simulink model "StampFly_StudentBlocks"  (R2026b)
settings: Solver=VariableStepAuto
undefined symbols (not defined in the file): Bottom, Official
(part 1 of 6)
settings Model: Creator=tyasukaw  LastModifiedBy=tyasukaw

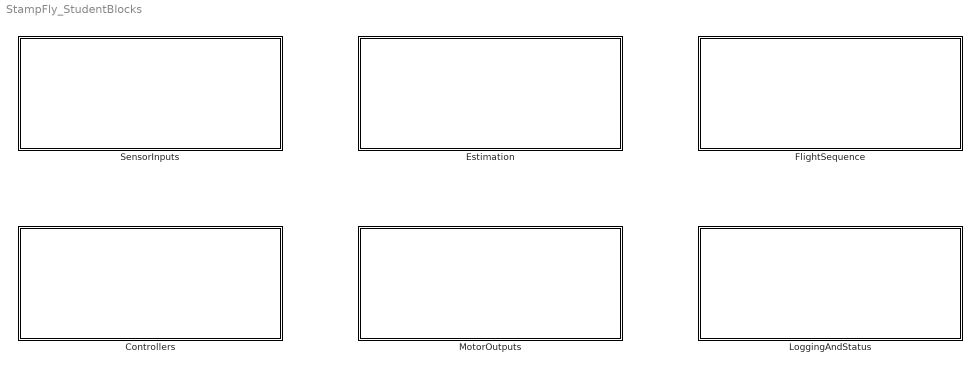
== system StampFly_StudentBlocks ==
  Controllers : Subsystem
      mask Display: disp('PID と指令生成')
  Estimation : Subsystem
      mask Display: disp('姿勢・高度の推定')
  FlightSequence : Subsystem
      mask Display: disp('飛行状態と離着陸')
  LoggingAndStatus : Subsystem
      mask Display: disp('記録・通信・LED')
  MotorOutputs : Subsystem
      mask Display: disp('PWM とモーター配分')
  SensorInputs : Subsystem
      mask Display: disp('センサー取得')

== system StampFly_StudentBlocks/Controllers ==
  AltitudePID : Subsystem  Description=高度誤差 → 上下速度指令
      mask Display: disp('高度 PID\n高度誤差 → 上下速度指令')
  PitchAnglePID : Subsystem  Description=角度誤差 → Pitch 角速度
      mask Display: disp('Pitch 姿勢 PID\n角度誤差 → Pitch 角速度')
  PitchRatePID : Subsystem  Description=角速度誤差 → モーター差分
      mask Display: disp('Pitch 角速度 PID\n角速度誤差 → モーター差分')
  RollAnglePID : Subsystem  Description=角度誤差 → Roll 角速度
      mask Display: disp('Roll 姿勢 PID\n角度誤差 → Roll 角速度')
  RollRatePID : Subsystem  Description=角速度誤差 → モーター差分
      mask Display: disp('Roll 角速度 PID\n角速度誤差 → モーター差分')
  SelectRateReference : Stateflow chart  Description=姿勢 PID / Sport / Flip  TreatAsAtomicUnit=on
      settings: AttributesFormatString=|
      | 角速度指令の選択
      | 姿勢 PID / Sport / Flip
  SelectVerticalReference : Stateflow chart  Description=自動高度 / 着陸 -0.15 m/s  TreatAsAtomicUnit=on
      settings: AttributesFormatString=|
      | 鉛直速度の指令選択
      | 自動高度 / 着陸 -0.15 m/s
  StickToAngleRate : Stateflow chart  Description=Stabilize / Sport / Flip  TreatAsAtomicUnit=on
      settings: AttributesFormatString=|
      | スティック → 姿勢・角速度
      | Stabilize / Sport / Flip
  TakeoffHoverControl400 : Subsystem  Description=飛行制御：目標値→誤差→高度PID/速度PID/姿勢PID/角速度PID→推力制限→ミキサー→8bit化。PIDの内部は標準演算ブロックです。
      mask Display: disp('TakeoffHoverControl400\nダブルクリックで内部を編集')
  ThrustCorrectionLimits : Stateflow chart  Description=基準推力 / フィルター / 上下限  TreatAsAtomicUnit=on
      settings: AttributesFormatString=|
      | 推力補正と制限
      | 基準推力 / フィルター / 上下限
  VerticalSpeedPID : Subsystem  Description=速度誤差 → 推力補正
      mask Display: disp('鉛直速度 PID\n速度誤差 → 推力補正')
  YawRatePID : Subsystem  Description=角速度誤差 → モーター差分
      mask Display: disp('Yaw 角速度 PID\n角速度誤差 → モーター差分')

== system StampFly_StudentBlocks/Estimation ==
  AltitudeKalman : Stateflow chart  Description=高度・鉛直速度・バイアス  TreatAsAtomicUnit=on
      settings: AttributesFormatString=|
      | 高度 Kalman 推定
      | 高度・鉛直速度・バイアス
  IMUAxisConversion : Stateflow chart  Description=BMI270 → 航空機座標  TreatAsAtomicUnit=on
      settings: AttributesFormatString=|
      | 軸・単位の変換
      | BMI270 → 航空機座標
  IMUBiasCalibration : Stateflow chart  Description=800サンプルでオフセット推定  TreatAsAtomicUnit=on
      settings: AttributesFormatString=|
      | 静止時の校正
      | 800サンプルでオフセット推定
  IMUFiltering : Stateflow chart  Description=校正値を引き一次フィルター  TreatAsAtomicUnit=on
      settings: AttributesFormatString=|
      | IMU フィルター
      | 校正値を引き一次フィルター
  MadgwickAttitude : Stateflow chart  Description=400 Hz / Roll・Pitch・Yaw  TreatAsAtomicUnit=on
      settings: AttributesFormatString=|
      | Madgwick 姿勢推定
      | 400 Hz / Roll・Pitch・Yaw
  SensorFlags : Stateflow chart  Description=距離異常・過加速度・低電圧  TreatAsAtomicUnit=on
      settings: AttributesFormatString=|
      | センサーの状態判定
      | 距離異常・過加速度・低電圧
  SensorProcessing400 : Subsystem  Description=センサー処理：軸変換、800点校正、フィルター、Madgwick、ToF保持/外れ値、高度Kalman、状態フラグを機能別に配置します。
      mask Display: disp('SensorProcessing400\nダブルクリックで内部を編集')
  ToFHoldOutlierFilter : Stateflow chart  Description=新着距離を判定 / 旧値を保持  TreatAsAtomicUnit=on
      settings: AttributesFormatString=|
      | ToF 保持・外れ値処理
      | 新着距離を判定 / 旧値を保持
  VerticalAcceleration : Stateflow chart  Description=重力成分を除去・フィルター  TreatAsAtomicUnit=on
      settings: AttributesFormatString=|
      | 鉛直加速度
      | 重力成分を除去・フィルター

== system StampFly_StudentBlocks/FlightSequence ==
  FinalizeFlightMode : Stateflow chart  Description=着陸終了・Flip・過加速度  TreatAsAtomicUnit=on
      settings: AttributesFormatString=|
      | 飛行モードの確定
      | 着陸終了・Flip・過加速度
  OfficialFlightSupervisor : Stateflow chart  TreatAsAtomicUnit=on
  OfficialFlipSequence : Stateflow chart  TreatAsAtomicUnit=on
  OfficialTakeoffHover400 : Subsystem  Description=全体制御：センサー前処理→推定→状態管理→離陸/高度/姿勢制御→4モーター指令。内部のブロックを個別に変更できます。
      mask Display: disp('姿勢・高度と飛行制御\n400 Hz / 内部を個別編集')
  TakeoffLandingCommand : Stateflow chart  Description=目標高度 / 基準推力 / カウンター  TreatAsAtomicUnit=on
      settings: AttributesFormatString=|
      | 離陸・着陸の指令
      | 目標高度 / 基準推力 / カウンター

== system StampFly_StudentBlocks/LoggingAndStatus ==
  CopiedLoggerSFI8_50 : MATLABSystem  Description=50 Hz SFI8記録：下向きToF距離[m]と状態、ToFValid=(距離>0かつ状態0)。ToFFreshは前回の記録から測定完了数が変化したかで判定。無効時も数値ペイロードと状態を保存し、UIは無効データをNaNで表示。Optical FlowはNaN/無効を保存。高度はSimulinkのKalman出力。  Priority=200  System=official.LoggerPacker50  SimulateUsing=Code generation
      mask Type: official.LoggerPacker50
  DataLogger50 : Subsystem  Description=50 Hz SFI8記録：下向きToF距離[m]と状態、ToFValid=(距離>0かつ状態0)。ToFFreshは前回の記録から測定完了数が変化したかで判定。無効時も数値ペイロードと状態を保存し、UIは無効データをNaNで表示。Optical FlowはNaN/無効を保存。高度はSimulinkのKalman出力。
      mask Display: disp('データロガー\n50 Hz / SFI8 / MAT 保存')
  ESPNowLogger50 : MATLABSystem  Description=ESP-NOWログ：コピーした受信機のログ形式を使います。送信キュー成功と相手の受信成功は別です。  Priority=221  System=imu.ESPNowIMUTx  Channel=uint8( 3 )  SimulateUsing=Code generation
      mask Type: imu.ESPNowIMUTx
  JoyStickTelemetry40 : Subsystem  Description=公式JoyStickへ40 Hzで姿勢・高度・電圧等を返信。前向きToFは無効で0を返信。
      mask Display: disp('JoyStick へ返信\n40 Hz / 公式パケット')
  OfficialJoyTelemetry40 : MATLABSystem  Description=公式JoyStickへ40 Hzで高度・電圧・姿勢・モード等を返信します。  Priority=240  System=official.RadioTelemetryWrite40  SimulateUsing=Code generation
      mask Type: official.RadioTelemetryWrite40
  OfficialTelemetryValues : Stateflow chart  TreatAsAtomicUnit=on
  QueuedUSBLogger50 : MATLABSystem  Description=USB送信：待ち時間0でキューへ投入し、別タスクから送信。PCのMATロガーで保存します。  Priority=220  System=official.USBLogger50  SimulateUsing=Code generation
      mask Type: official.USBLogger50
  StatusIndicators400 : Stateflow chart  TreatAsAtomicUnit=on
  StatusOutputs400 : Subsystem  Description=LED・ブザー・ボタン｜表示判断はモデル、出力はドライバー
      mask Display: disp('LED とブザー\n400 Hz 判断 / 送出キュー')
  StatusWrite400 : MATLABSystem  System=official.StatusWrite400  SimulateUsing=Code generation
      mask Type: official.StatusWrite400

== system StampFly_StudentBlocks/MotorOutputs ==
  MotorMixerFilter8bit : Subsystem  Description=4ch / Duty 0〜0.95 / 8 bit
      mask Display: disp('モーター配分・フィルター\n4ch / Duty 0〜0.95 / 8 bit')
  MotorOutputs400 : Subsystem  Description=モーター出力｜400 Hz更新・150 kHz／8 bit
      mask Display: disp('モーター出力\n150 kHz / 8 bit / 出力ゼロ')
  PWM150kHz8bit : MATLABSystem  Description=モーター書き込み：150 kHz指定、8 bit、FR/FL/RR/RL=GPIO42/5/41/10。実機ベンチではAllowMotorOutput=falseかつEnable=false、出力0です。  Priority=100  System=official.MotorPWM400  SampleTime=Official.Step  AllowMotorOutput=false  SimulateUsing=Code generation
      mask Type: official.MotorPWM400

== system StampFly_StudentBlocks/SensorInputs ==
  BMI270_400 : MATLABSystem  Description=BMI270取得：加速度[m/s²]・角速度[rad/s]・温度・新規データ有無。センサーODRは400 Hzです。  Priority=2  System=stampfly.BMI270IMU  SampleTime=Official.Step  SimulateUsing=Code generation
      mask Type: stampfly.BMI270IMU
  Battery400 : MATLABSystem  Description=電池電圧取得：毎周期読み出しを試みます。ToFがI2C使用中なら最新保持値とReadValid=0を返します。  Priority=4  System=official.Battery400  SampleTime=Official.Step  SimulateUsing=Code generation
      mask Type: official.Battery400
  OfficialJoystick400 : MATLABSystem  Description=JoyStick取得：公式ESP-NOWパケットからスティック、アームボタン、通信状態、姿勢リセット要求を取得します。  Priority=5  System=official.Joystick400  SampleTime=Official.Step  Channel=uint8( 3 )  SimulateUsing=Code generation
      mask Type: official.Joystick400
  ToFReadyPoll400 : MATLABSystem  Description=下向きToF：Medium、33 ms。起動時のStartMeasurementは1回。dcnt>14とready割り込みでcore0へ読み出しを要求し、400 Hz側は待たず最新結果を取得。状態0の最遠対象[mm]、新着フラグ、測定状態を出力。前向きToFはXSHUT=LOWで無効。  Priority=3  System=official.BottomToF400  Sensor=Bottom (0x29)  I2CAddress=uint8( 41 )  SampleTime=Official.Step  DistanceMode=Auto (bottom Medium / front Long)  TimingBudget=20  PerformBringUp=on  TargetSelect=Auto (bottom Farthest / front Nearest)  SimulateUsing=Code generation
      mask Type: official.BottomToF400
  UserButton400 : MATLABSystem  System=official.UserButton400  SimulateUsing=Code generation
      mask Type: official.UserButton400

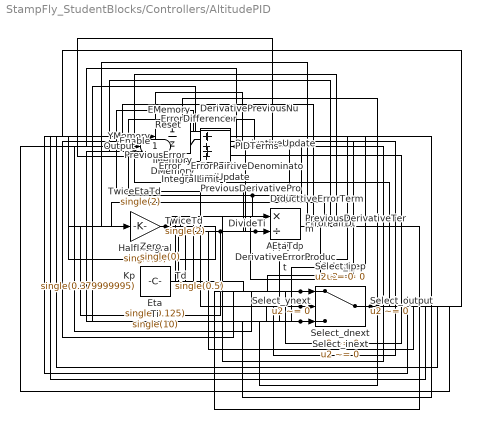
== system StampFly_StudentBlocks/Controllers/AltitudePID ==
  Error : Inport
  Dt : Inport  Port=2
  Enable : Inport  Port=3
  Reset : Inport  Port=4
  PreviousError : Inport  Port=5
  ApplyKp : Product
  DMemory : UnitDelay  InitialCondition=single(0)  SampleTime=Official.Step
  DerivativeDenominator : Sum
  DerivativeErrorProduct : Product
  DerivativeErrorTerm : Product  Inputs=*/
  DerivativePreviousNumerator : Sum  Inputs=+-
  DerivativeUpdate : Sum
  DivideTi : Product  Inputs=*/
  EMemory : UnitDelay  InitialCondition=single(0)  SampleTime=Official.Step
  ErrorDifference : Sum  Inputs=+-
  ErrorPair : Sum
  ErrorPairDt : Product
  Eta : Constant  Value=single(0.125)
  EtaTd : Product
  HalfIntegral : Gain  Gain=single(.5)
  IMemory : UnitDelay  InitialCondition=single(0)  SampleTime=Official.Step
  IntegralLimit : Saturate  UpperLimit=single(30000)  LowerLimit=single(-30000)
  IntegralUpdate : Sum
  Kp : Constant  Value=single(0.379999995)
  PIDTerms : Sum  Inputs=+++
  PreviousDerivativeProduct : Product
  PreviousDerivativeTerm : Product  Inputs=*/
  Select_dnext : Switch  Criteria=u2 ~= 0  SaturateOnIntegerOverflow=off  InputSameDT=off
  Select_dp : Switch  Criteria=u2 ~= 0  SaturateOnIntegerOverflow=off  InputSameDT=off
  Select_enext : Switch  Criteria=u2 ~= 0  SaturateOnIntegerOverflow=off  InputSameDT=off
  Select_ep : Switch  Criteria=u2 ~= 0  SaturateOnIntegerOverflow=off  InputSameDT=off
  Select_inext : Switch  Criteria=u2 ~= 0  SaturateOnIntegerOverflow=off  InputSameDT=off
  Select_ip : Switch  Criteria=u2 ~= 0  SaturateOnIntegerOverflow=off  InputSameDT=off
  Select_output : Switch  Criteria=u2 ~= 0  SaturateOnIntegerOverflow=off  InputSameDT=off
  Select_ynext : Switch  Criteria=u2 ~= 0  SaturateOnIntegerOverflow=off  InputSameDT=off
  Td : Constant  Value=single(0.5)
  Ti : Constant  Value=single(10)
  TwiceEtaTd : Gain  Gain=single(2)
  TwiceTd : Gain  Gain=single(2)
  YMemory : UnitDelay  InitialCondition=single(0)  SampleTime=Official.Step
  Zero : Constant  Value=single(0)
  Output : Outport
  wires:
  Select_output/1 -> Output/1
  Select_ynext/1 -> YMemory/1
  YMemory/1 -> Select_ynext/3, Select_output/3
  ApplyKp/1 -> Select_ynext/1, Select_output/1
  Select_enext/1 -> EMemory/1
  Select_dnext/1 -> DMemory/1
  Select_inext/1 -> IMemory/1
  Enable/1 -> Select_inext/2, Select_dnext/2, Select_enext/2, Select_ynext/2, Select_output/2
  PIDTerms/1 -> ApplyKp/2
  Kp/1 -> ApplyKp/1
  DerivativeUpdate/1 -> PIDTerms/3, Select_dnext/1
  IntegralLimit/1 -> PIDTerms/2, Select_inext/1
  DerivativeErrorTerm/1 -> DerivativeUpdate/2
  PreviousDerivativeTerm/1 -> DerivativeUpdate/1
  DerivativeErrorProduct/1 -> DerivativeErrorTerm/1
  ErrorDifference/1 -> DerivativeErrorProduct/2
  TwiceTd/1 -> DerivativeErrorProduct/1
  DerivativeDenominator/1 -> PreviousDerivativeTerm/2, DerivativeErrorTerm/2
  PreviousDerivativeProduct/1 -> PreviousDerivativeTerm/1
  Select_dp/1 -> PreviousDerivativeProduct/2, Select_dnext/3
  DerivativePreviousNumerator/1 -> PreviousDerivativeProduct/1
  TwiceEtaTd/1 -> DerivativePreviousNumerator/1, DerivativeDenominator/1
  EtaTd/1 -> TwiceEtaTd/1
  Td/1 -> EtaTd/2, TwiceTd/1
  Eta/1 -> EtaTd/1
  IntegralUpdate/1 -> IntegralLimit/1
  DivideTi/1 -> IntegralUpdate/2
  Select_ip/1 -> Select_inext/3, IntegralUpdate/1
  Ti/1 -> DivideTi/2
  HalfIntegral/1 -> DivideTi/1
  ErrorPairDt/1 -> HalfIntegral/1
  ErrorPair/1 -> ErrorPairDt/2
  Dt/1 -> ErrorPairDt/1, DerivativeDenominator/2, DerivativePreviousNumerator/2
  Select_ep/1 -> Select_enext/3, ErrorPair/2, ErrorDifference/2
  Error/1 -> ErrorPair/1, ErrorDifference/1, PIDTerms/1, Select_enext/1
  EMemory/1 -> Select_ep/3
  PreviousError/1 -> Select_ep/1
  DMemory/1 -> Select_dp/3
  IMemory/1 -> Select_ip/3
  Reset/1 -> Select_ip/2, Select_dp/2, Select_ep/2
  Zero/1 -> Select_ip/1, Select_dp/1

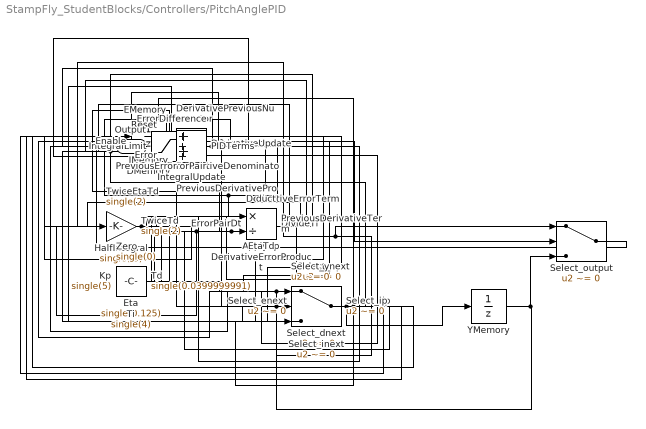
== system StampFly_StudentBlocks/Controllers/PitchAnglePID ==
  Error : Inport
  Dt : Inport  Port=2
  Enable : Inport  Port=3
  Reset : Inport  Port=4
  PreviousError : Inport  Port=5
  ApplyKp : Product
  DMemory : UnitDelay  InitialCondition=single(0)  SampleTime=Official.Step
  DerivativeDenominator : Sum
  DerivativeErrorProduct : Product
  DerivativeErrorTerm : Product  Inputs=*/
  DerivativePreviousNumerator : Sum  Inputs=+-
  DerivativeUpdate : Sum
  DivideTi : Product  Inputs=*/
  EMemory : UnitDelay  InitialCondition=single(0)  SampleTime=Official.Step
  ErrorDifference : Sum  Inputs=+-
  ErrorPair : Sum
  ErrorPairDt : Product
  Eta : Constant  Value=single(0.125)
  EtaTd : Product
  HalfIntegral : Gain  Gain=single(.5)
  IMemory : UnitDelay  InitialCondition=single(0)  SampleTime=Official.Step
  IntegralLimit : Saturate  UpperLimit=single(30000)  LowerLimit=single(-30000)
  IntegralUpdate : Sum
  Kp : Constant  Value=single(5)
  PIDTerms : Sum  Inputs=+++
  PreviousDerivativeProduct : Product
  PreviousDerivativeTerm : Product  Inputs=*/
  Select_dnext : Switch  Criteria=u2 ~= 0  SaturateOnIntegerOverflow=off  InputSameDT=off
  Select_dp : Switch  Criteria=u2 ~= 0  SaturateOnIntegerOverflow=off  InputSameDT=off
  Select_enext : Switch  Criteria=u2 ~= 0  SaturateOnIntegerOverflow=off  InputSameDT=off
  Select_ep : Switch  Criteria=u2 ~= 0  SaturateOnIntegerOverflow=off  InputSameDT=off
  Select_inext : Switch  Criteria=u2 ~= 0  SaturateOnIntegerOverflow=off  InputSameDT=off
  Select_ip : Switch  Criteria=u2 ~= 0  SaturateOnIntegerOverflow=off  InputSameDT=off
  Select_output : Switch  Criteria=u2 ~= 0  SaturateOnIntegerOverflow=off  InputSameDT=off
  Select_ynext : Switch  Criteria=u2 ~= 0  SaturateOnIntegerOverflow=off  InputSameDT=off
  Td : Constant  Value=single(0.0399999991)
  Ti : Constant  Value=single(4)
  TwiceEtaTd : Gain  Gain=single(2)
  TwiceTd : Gain  Gain=single(2)
  YMemory : UnitDelay  InitialCondition=single(0)  SampleTime=Official.Step
  Zero : Constant  Value=single(0)
  Output : Outport
  wires:
  Enable/1 -> Select_output/2, Select_inext/2, Select_dnext/2, Select_enext/2, Select_ynext/2
  ApplyKp/1 -> Select_ynext/1, Select_output/1
  YMemory/1 -> Select_ynext/3, Select_output/3
  Select_ynext/1 -> YMemory/1
  Select_output/1 -> Output/1
  Select_enext/1 -> EMemory/1
  Select_dnext/1 -> DMemory/1
  Select_inext/1 -> IMemory/1
  PIDTerms/1 -> ApplyKp/2
  Kp/1 -> ApplyKp/1
  DerivativeUpdate/1 -> PIDTerms/3, Select_dnext/1
  IntegralLimit/1 -> PIDTerms/2, Select_inext/1
  DerivativeErrorTerm/1 -> DerivativeUpdate/2
  PreviousDerivativeTerm/1 -> DerivativeUpdate/1
  DerivativeErrorProduct/1 -> DerivativeErrorTerm/1
  ErrorDifference/1 -> DerivativeErrorProduct/2
  TwiceTd/1 -> DerivativeErrorProduct/1
  DerivativeDenominator/1 -> PreviousDerivativeTerm/2, DerivativeErrorTerm/2
  PreviousDerivativeProduct/1 -> PreviousDerivativeTerm/1
  Select_dp/1 -> PreviousDerivativeProduct/2, Select_dnext/3
  DerivativePreviousNumerator/1 -> PreviousDerivativeProduct/1
  TwiceEtaTd/1 -> DerivativePreviousNumerator/1, DerivativeDenominator/1
  EtaTd/1 -> TwiceEtaTd/1
  Td/1 -> EtaTd/2, TwiceTd/1
  Eta/1 -> EtaTd/1
  IntegralUpdate/1 -> IntegralLimit/1
  DivideTi/1 -> IntegralUpdate/2
  Select_ip/1 -> Select_inext/3, IntegralUpdate/1
  Ti/1 -> DivideTi/2
  HalfIntegral/1 -> DivideTi/1
  ErrorPairDt/1 -> HalfIntegral/1
  ErrorPair/1 -> ErrorPairDt/2
  Dt/1 -> ErrorPairDt/1, DerivativeDenominator/2, DerivativePreviousNumerator/2
  Select_ep/1 -> Select_enext/3, ErrorPair/2, ErrorDifference/2
  Error/1 -> ErrorPair/1, ErrorDifference/1, PIDTerms/1, Select_enext/1
  EMemory/1 -> Select_ep/3
  PreviousError/1 -> Select_ep/1
  DMemory/1 -> Select_dp/3
  IMemory/1 -> Select_ip/3
  Reset/1 -> Select_ip/2, Select_dp/2, Select_ep/2
  Zero/1 -> Select_ip/1, Select_dp/1

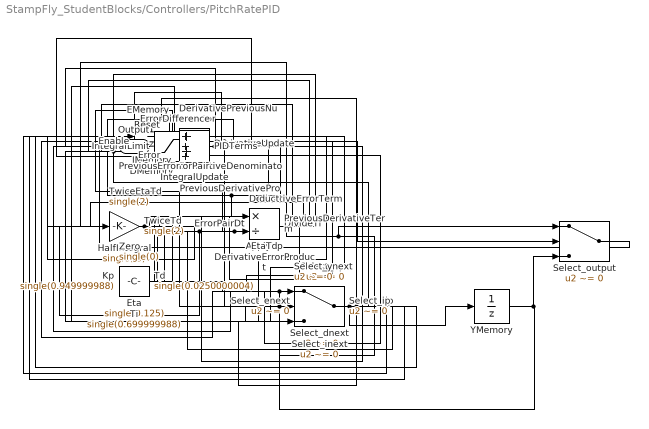
== system StampFly_StudentBlocks/Controllers/PitchRatePID ==
  Error : Inport
  Dt : Inport  Port=2
  Enable : Inport  Port=3
  Reset : Inport  Port=4
  PreviousError : Inport  Port=5
  ApplyKp : Product
  DMemory : UnitDelay  InitialCondition=single(0)  SampleTime=Official.Step
  DerivativeDenominator : Sum
  DerivativeErrorProduct : Product
  DerivativeErrorTerm : Product  Inputs=*/
  DerivativePreviousNumerator : Sum  Inputs=+-
  DerivativeUpdate : Sum
  DivideTi : Product  Inputs=*/
  EMemory : UnitDelay  InitialCondition=single(0)  SampleTime=Official.Step
  ErrorDifference : Sum  Inputs=+-
  ErrorPair : Sum
  ErrorPairDt : Product
  Eta : Constant  Value=single(0.125)
  EtaTd : Product
  HalfIntegral : Gain  Gain=single(.5)
  IMemory : UnitDelay  InitialCondition=single(0)  SampleTime=Official.Step
  IntegralLimit : Saturate  UpperLimit=single(30000)  LowerLimit=single(-30000)
  IntegralUpdate : Sum
  Kp : Constant  Value=single(0.949999988)
  PIDTerms : Sum  Inputs=+++
  PreviousDerivativeProduct : Product
  PreviousDerivativeTerm : Product  Inputs=*/
  Select_dnext : Switch  Criteria=u2 ~= 0  SaturateOnIntegerOverflow=off  InputSameDT=off
  Select_dp : Switch  Criteria=u2 ~= 0  SaturateOnIntegerOverflow=off  InputSameDT=off
  Select_enext : Switch  Criteria=u2 ~= 0  SaturateOnIntegerOverflow=off  InputSameDT=off
  Select_ep : Switch  Criteria=u2 ~= 0  SaturateOnIntegerOverflow=off  InputSameDT=off
  Select_inext : Switch  Criteria=u2 ~= 0  SaturateOnIntegerOverflow=off  InputSameDT=off
  Select_ip : Switch  Criteria=u2 ~= 0  SaturateOnIntegerOverflow=off  InputSameDT=off
  Select_output : Switch  Criteria=u2 ~= 0  SaturateOnIntegerOverflow=off  InputSameDT=off
  Select_ynext : Switch  Criteria=u2 ~= 0  SaturateOnIntegerOverflow=off  InputSameDT=off
  Td : Constant  Value=single(0.0250000004)
  Ti : Constant  Value=single(0.699999988)
  TwiceEtaTd : Gain  Gain=single(2)
  TwiceTd : Gain  Gain=single(2)
  YMemory : UnitDelay  InitialCondition=single(0)  SampleTime=Official.Step
  Zero : Constant  Value=single(0)
  Output : Outport
  wires:
  Enable/1 -> Select_output/2, Select_inext/2, Select_dnext/2, Select_enext/2, Select_ynext/2
  ApplyKp/1 -> Select_ynext/1, Select_output/1
  YMemory/1 -> Select_ynext/3, Select_output/3
  Select_ynext/1 -> YMemory/1
  Select_output/1 -> Output/1
  Select_enext/1 -> EMemory/1
  Select_dnext/1 -> DMemory/1
  Select_inext/1 -> IMemory/1
  PIDTerms/1 -> ApplyKp/2
  Kp/1 -> ApplyKp/1
  DerivativeUpdate/1 -> PIDTerms/3, Select_dnext/1
  IntegralLimit/1 -> PIDTerms/2, Select_inext/1
  DerivativeErrorTerm/1 -> DerivativeUpdate/2
  PreviousDerivativeTerm/1 -> DerivativeUpdate/1
  DerivativeErrorProduct/1 -> DerivativeErrorTerm/1
  ErrorDifference/1 -> DerivativeErrorProduct/2
  TwiceTd/1 -> DerivativeErrorProduct/1
  DerivativeDenominator/1 -> PreviousDerivativeTerm/2, DerivativeErrorTerm/2
  PreviousDerivativeProduct/1 -> PreviousDerivativeTerm/1
  Select_dp/1 -> PreviousDerivativeProduct/2, Select_dnext/3
  DerivativePreviousNumerator/1 -> PreviousDerivativeProduct/1
  TwiceEtaTd/1 -> DerivativePreviousNumerator/1, DerivativeDenominator/1
  EtaTd/1 -> TwiceEtaTd/1
  Td/1 -> EtaTd/2, TwiceTd/1
  Eta/1 -> EtaTd/1
  IntegralUpdate/1 -> IntegralLimit/1
  DivideTi/1 -> IntegralUpdate/2
  Select_ip/1 -> Select_inext/3, IntegralUpdate/1
  Ti/1 -> DivideTi/2
  HalfIntegral/1 -> DivideTi/1
  ErrorPairDt/1 -> HalfIntegral/1
  ErrorPair/1 -> ErrorPairDt/2
  Dt/1 -> ErrorPairDt/1, DerivativeDenominator/2, DerivativePreviousNumerator/2
  Select_ep/1 -> Select_enext/3, ErrorPair/2, ErrorDifference/2
  Error/1 -> ErrorPair/1, ErrorDifference/1, PIDTerms/1, Select_enext/1
  EMemory/1 -> Select_ep/3
  PreviousError/1 -> Select_ep/1
  DMemory/1 -> Select_dp/3
  IMemory/1 -> Select_ip/3
  Reset/1 -> Select_ip/2, Select_dp/2, Select_ep/2
  Zero/1 -> Select_ip/1, Select_dp/1

== system StampFly_StudentBlocks/Controllers/RollAnglePID ==
  Error : Inport
  Dt : Inport  Port=2
  Enable : Inport  Port=3
  Reset : Inport  Port=4
  PreviousError : Inport  Port=5
  ApplyKp : Product
  DMemory : UnitDelay  InitialCondition=single(0)  SampleTime=Official.Step
  DerivativeDenominator : Sum
  DerivativeErrorProduct : Product
  DerivativeErrorTerm : Product  Inputs=*/
  DerivativePreviousNumerator : Sum  Inputs=+-
  DerivativeUpdate : Sum
  DivideTi : Product  Inputs=*/
  EMemory : UnitDelay  InitialCondition=single(0)  SampleTime=Official.Step
  ErrorDifference : Sum  Inputs=+-
  ErrorPair : Sum
  ErrorPairDt : Product
  Eta : Constant  Value=single(0.125)
  EtaTd : Product
  HalfIntegral : Gain  Gain=single(.5)
  IMemory : UnitDelay  InitialCondition=single(0)  SampleTime=Official.Step
  IntegralLimit : Saturate  UpperLimit=single(30000)  LowerLimit=single(-30000)
  IntegralUpdate : Sum
  Kp : Constant  Value=single(5)
  PIDTerms : Sum  Inputs=+++
  PreviousDerivativeProduct : Product
  PreviousDerivativeTerm : Product  Inputs=*/
  Select_dnext : Switch  Criteria=u2 ~= 0  SaturateOnIntegerOverflow=off  InputSameDT=off
  Select_dp : Switch  Criteria=u2 ~= 0  SaturateOnIntegerOverflow=off  InputSameDT=off
  Select_enext : Switch  Criteria=u2 ~= 0  SaturateOnIntegerOverflow=off  InputSameDT=off
  Select_ep : Switch  Criteria=u2 ~= 0  SaturateOnIntegerOverflow=off  InputSameDT=off
  Select_inext : Switch  Criteria=u2 ~= 0  SaturateOnIntegerOverflow=off  InputSameDT=off
  Select_ip : Switch  Criteria=u2 ~= 0  SaturateOnIntegerOverflow=off  InputSameDT=off
  Select_output : Switch  Criteria=u2 ~= 0  SaturateOnIntegerOverflow=off  InputSameDT=off
  Select_ynext : Switch  Criteria=u2 ~= 0  SaturateOnIntegerOverflow=off  InputSameDT=off
  Td : Constant  Value=single(0.0399999991)
  Ti : Constant  Value=single(4)
  TwiceEtaTd : Gain  Gain=single(2)
  TwiceTd : Gain  Gain=single(2)
  YMemory : UnitDelay  InitialCondition=single(0)  SampleTime=Official.Step
  Zero : Constant  Value=single(0)
  Output : Outport
  wires:
  Enable/1 -> Select_output/2, Select_inext/2, Select_dnext/2, Select_enext/2, Select_ynext/2
  ApplyKp/1 -> Select_ynext/1, Select_output/1
  YMemory/1 -> Select_ynext/3, Select_output/3
  Select_ynext/1 -> YMemory/1
  Select_output/1 -> Output/1
  Select_enext/1 -> EMemory/1
  Select_dnext/1 -> DMemory/1
  Select_inext/1 -> IMemory/1
  PIDTerms/1 -> ApplyKp/2
  Kp/1 -> ApplyKp/1
  DerivativeUpdate/1 -> PIDTerms/3, Select_dnext/1
  IntegralLimit/1 -> PIDTerms/2, Select_inext/1
  DerivativeErrorTerm/1 -> DerivativeUpdate/2
  PreviousDerivativeTerm/1 -> DerivativeUpdate/1
  DerivativeErrorProduct/1 -> DerivativeErrorTerm/1
  ErrorDifference/1 -> DerivativeErrorProduct/2
  TwiceTd/1 -> DerivativeErrorProduct/1
  DerivativeDenominator/1 -> PreviousDerivativeTerm/2, DerivativeErrorTerm/2
  PreviousDerivativeProduct/1 -> PreviousDerivativeTerm/1
  Select_dp/1 -> PreviousDerivativeProduct/2, Select_dnext/3
  DerivativePreviousNumerator/1 -> PreviousDerivativeProduct/1
  TwiceEtaTd/1 -> DerivativePreviousNumerator/1, DerivativeDenominator/1
  EtaTd/1 -> TwiceEtaTd/1
  Td/1 -> EtaTd/2, TwiceTd/1
  Eta/1 -> EtaTd/1
  IntegralUpdate/1 -> IntegralLimit/1
  DivideTi/1 -> IntegralUpdate/2
  Select_ip/1 -> Select_inext/3, IntegralUpdate/1
  Ti/1 -> DivideTi/2
  HalfIntegral/1 -> DivideTi/1
  ErrorPairDt/1 -> HalfIntegral/1
  ErrorPair/1 -> ErrorPairDt/2
  Dt/1 -> ErrorPairDt/1, DerivativeDenominator/2, DerivativePreviousNumerator/2
  Select_ep/1 -> Select_enext/3, ErrorPair/2, ErrorDifference/2
  Error/1 -> ErrorPair/1, ErrorDifference/1, PIDTerms/1, Select_enext/1
  EMemory/1 -> Select_ep/3
  PreviousError/1 -> Select_ep/1
  DMemory/1 -> Select_dp/3
  IMemory/1 -> Select_ip/3
  Reset/1 -> Select_ip/2, Select_dp/2, Select_ep/2
  Zero/1 -> Select_ip/1, Select_dp/1

== system StampFly_StudentBlocks/Controllers/RollRatePID ==
  Error : Inport
  Dt : Inport  Port=2
  Enable : Inport  Port=3
  Reset : Inport  Port=4
  PreviousError : Inport  Port=5
  ApplyKp : Product
  DMemory : UnitDelay  InitialCondition=single(0)  SampleTime=Official.Step
  DerivativeDenominator : Sum
  DerivativeErrorProduct : Product
  DerivativeErrorTerm : Product  Inputs=*/
  DerivativePreviousNumerator : Sum  Inputs=+-
  DerivativeUpdate : Sum
  DivideTi : Product  Inputs=*/
  EMemory : UnitDelay  InitialCondition=single(0)  SampleTime=Official.Step
  ErrorDifference : Sum  Inputs=+-
  ErrorPair : Sum
  ErrorPairDt : Product
  Eta : Constant  Value=single(0.125)
  EtaTd : Product
  HalfIntegral : Gain  Gain=single(.5)
  IMemory : UnitDelay  InitialCondition=single(0)  SampleTime=Official.Step
  IntegralLimit : Saturate  UpperLimit=single(30000)  LowerLimit=single(-30000)
  IntegralUpdate : Sum
  Kp : Constant  Value=single(0.649999976)
  PIDTerms : Sum  Inputs=+++
  PreviousDerivativeProduct : Product
  PreviousDerivativeTerm : Product  Inputs=*/
  Select_dnext : Switch  Criteria=u2 ~= 0  SaturateOnIntegerOverflow=off  InputSameDT=off
  Select_dp : Switch  Criteria=u2 ~= 0  SaturateOnIntegerOverflow=off  InputSameDT=off
  Select_enext : Switch  Criteria=u2 ~= 0  SaturateOnIntegerOverflow=off  InputSameDT=off
  Select_ep : Switch  Criteria=u2 ~= 0  SaturateOnIntegerOverflow=off  InputSameDT=off
  Select_inext : Switch  Criteria=u2 ~= 0  SaturateOnIntegerOverflow=off  InputSameDT=off
  Select_ip : Switch  Criteria=u2 ~= 0  SaturateOnIntegerOverflow=off  InputSameDT=off
  Select_output : Switch  Criteria=u2 ~= 0  SaturateOnIntegerOverflow=off  InputSameDT=off
  Select_ynext : Switch  Criteria=u2 ~= 0  SaturateOnIntegerOverflow=off  InputSameDT=off
  Td : Constant  Value=single(0.00999999978)
  Ti : Constant  Value=single(0.699999988)
  TwiceEtaTd : Gain  Gain=single(2)
  TwiceTd : Gain  Gain=single(2)
  YMemory : UnitDelay  InitialCondition=single(0)  SampleTime=Official.Step
  Zero : Constant  Value=single(0)
  Output : Outport
  wires:
  Enable/1 -> Select_output/2, Select_inext/2, Select_dnext/2, Select_enext/2, Select_ynext/2
  ApplyKp/1 -> Select_ynext/1, Select_output/1
  YMemory/1 -> Select_ynext/3, Select_output/3
  Select_ynext/1 -> YMemory/1
  Select_output/1 -> Output/1
  Select_enext/1 -> EMemory/1
  Select_dnext/1 -> DMemory/1
  Select_inext/1 -> IMemory/1
  PIDTerms/1 -> ApplyKp/2
  Kp/1 -> ApplyKp/1
  DerivativeUpdate/1 -> PIDTerms/3, Select_dnext/1
  IntegralLimit/1 -> PIDTerms/2, Select_inext/1
  DerivativeErrorTerm/1 -> DerivativeUpdate/2
  PreviousDerivativeTerm/1 -> DerivativeUpdate/1
  DerivativeErrorProduct/1 -> DerivativeErrorTerm/1
  ErrorDifference/1 -> DerivativeErrorProduct/2
  TwiceTd/1 -> DerivativeErrorProduct/1
  DerivativeDenominator/1 -> PreviousDerivativeTerm/2, DerivativeErrorTerm/2
  PreviousDerivativeProduct/1 -> PreviousDerivativeTerm/1
  Select_dp/1 -> PreviousDerivativeProduct/2, Select_dnext/3
  DerivativePreviousNumerator/1 -> PreviousDerivativeProduct/1
  TwiceEtaTd/1 -> DerivativePreviousNumerator/1, DerivativeDenominator/1
  EtaTd/1 -> TwiceEtaTd/1
  Td/1 -> EtaTd/2, TwiceTd/1
  Eta/1 -> EtaTd/1
  IntegralUpdate/1 -> IntegralLimit/1
  DivideTi/1 -> IntegralUpdate/2
  Select_ip/1 -> Select_inext/3, IntegralUpdate/1
  Ti/1 -> DivideTi/2
  HalfIntegral/1 -> DivideTi/1
  ErrorPairDt/1 -> HalfIntegral/1
  ErrorPair/1 -> ErrorPairDt/2
  Dt/1 -> ErrorPairDt/1, DerivativeDenominator/2, DerivativePreviousNumerator/2
  Select_ep/1 -> Select_enext/3, ErrorPair/2, ErrorDifference/2
  Error/1 -> ErrorPair/1, ErrorDifference/1, PIDTerms/1, Select_enext/1
  EMemory/1 -> Select_ep/3
  PreviousError/1 -> Select_ep/1
  DMemory/1 -> Select_dp/3
  IMemory/1 -> Select_ip/3
  Reset/1 -> Select_ip/2, Select_dp/2, Select_ep/2
  Zero/1 -> Select_ip/1, Select_dp/1

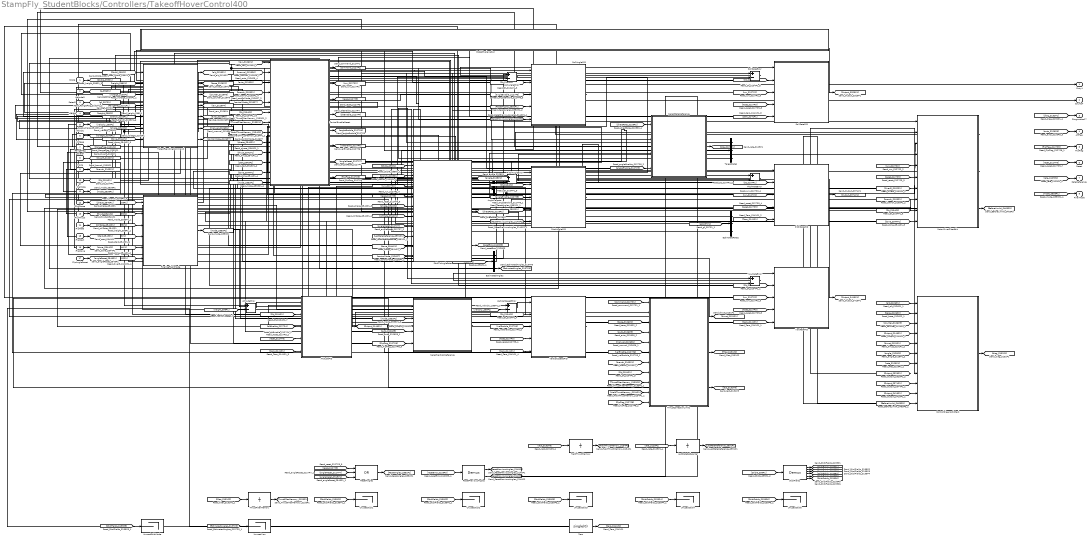
== system StampFly_StudentBlocks/Controllers/TakeoffHoverControl400 ==
  Stick6 : Inport
  Attitude3 : Inport  Port=2
  Rates3 : Inport  Port=3
  Height : Inport  Port=4
  Velocity : Inport  Port=5
  Voltage : Inport  Port=6
  RangeFlag : Inport  Port=7
  OverG : Inport  Port=8
  Mode : Inport  Port=9
  Dt : Inport  Port=10
  PreMode : Inport  Port=11
  FlipPhase : Inport  Port=12
  FlipThrust : Inport  Port=13
  FlipRate : Inport  Port=14
  FlipStart : Inport  Port=15
  FlipDone : Inport  Port=16
  FlipAngleReset : Inport  Port=17
  AltitudeError : Sum  Inputs=+-
  AltitudePID : Subsystem  Description=高度誤差 → 上下速度指令
      mask Display: disp('高度 PID\n高度誤差 → 上下速度指令')
  AngleTargets : Demux  Outputs=2
  ControlDiagnosticPack : Stateflow chart  Description=目標・補正量・配分前出力  TreatAsAtomicUnit=on
      settings: AttributesFormatString=|
      | 制御の診断信号
      | 目標・補正量・配分前出力
  ControlEnableReset : Stateflow chart  Description=各 PID の実行条件を決める  TreatAsAtomicUnit=on
      settings: AttributesFormatString=|
      | 制御の有効化とリセット
      | 各 PID の実行条件を決める
  EstimatedAngles : Demux  Outputs=3
  EstimatedRates : Demux  Outputs=3
  FinalizeFlightMode : Stateflow chart  Description=着陸終了・Flip・過加速度  TreatAsAtomicUnit=on
      settings: AttributesFormatString=|
      | 飛行モードの確定
      | 着陸終了・Flip・過加速度
  HeldThrustMemory : UnitDelay  InitialCondition=single(0)  SampleTime=Official.Step
  LastRateReference : UnitDelay  InitialCondition=zeros(3,1,'single')  SampleTime=Official.Step
  ModelExplanation : Subsystem  Description=400 Hz の制御：高度 PID → 鉛直速度 PID → 共通推力。姿勢 PID → 角速度 PID → 4モーター配分。各 PID 内部は Sum / Gain / Unit Delay。共有の実行・リセット条件は名前付き信号で接続。
      mask Display: disp('説明\n400 Hz の制御：高度 PID → 鉛直速度 PID → 共通推力。姿勢 PID → 角速度 PID → 4モーター配分。各 PID 内部は Sum / Gain / Unit Delay。共有の実行・リセット条件は名前付き信号で接続。')
  MotorMixerFilter8bit : Subsystem  Description=4ch / Duty 0〜0.95 / 8 bit
      mask Display: disp('モーター配分・フィルター\n4ch / Duty 0〜0.95 / 8 bit')
  PitchAngleError : Sum  Inputs=+-
  PitchAnglePID : Subsystem  Description=角度誤差 → Pitch 角速度
      mask Display: disp('Pitch 姿勢 PID\n角度誤差 → Pitch 角速度')
  PitchRateError : Sum  Inputs=+-
  PitchRatePID : Subsystem  Description=角速度誤差 → モーター差分
      mask Display: disp('Pitch 角速度 PID\n角速度誤差 → モーター差分')
  ResetAngles : Logic  Operator=OR  Inputs=3  AllPortsSameDT=off  OutDataTypeStr=boolean
  ResetPreviousAngles : Demux  Outputs=2
  RollAngleError : Sum  Inputs=+-
  RollAnglePID : Subsystem  Description=角度誤差 → Roll 角速度
      mask Display: disp('Roll 姿勢 PID\n角度誤差 → Roll 角速度')
  RollRateError : Sum  Inputs=+-
  RollRatePID : Subsystem  Description=角速度誤差 → モーター差分
      mask Display: disp('Roll 角速度 PID\n角速度誤差 → モーター差分')
  SelectRateReference : Stateflow chart  Description=姿勢 PID / Sport / Flip  TreatAsAtomicUnit=on
      settings: AttributesFormatString=|
      | 角速度指令の選択
      | 姿勢 PID / Sport / Flip
  SelectVerticalReference : Stateflow chart  Description=自動高度 / 着陸 -0.15 m/s  TreatAsAtomicUnit=on
      settings: AttributesFormatString=|
      | 鉛直速度の指令選択
      | 自動高度 / 着陸 -0.15 m/s
  StickFields : Demux  Outputs=6
  StickToAngleRate : Stateflow chart  Description=Stabilize / Sport / Flip  TreatAsAtomicUnit=on
      settings: AttributesFormatString=|
      | スティック → 姿勢・角速度
      | Stabilize / Sport / Flip
  TakeoffLandingCommand : Stateflow chart  Description=目標高度 / 基準推力 / カウンター  TreatAsAtomicUnit=on
      settings: AttributesFormatString=|
      | 離陸・着陸の指令
      | 目標高度 / 基準推力 / カウンター
  TargetRates : Demux  Outputs=3
  ThrustCorrectionLimits : Stateflow chart  Description=基準推力 / フィルター / 上下限  TreatAsAtomicUnit=on
      settings: AttributesFormatString=|
      | 推力補正と制限
      | 基準推力 / フィルター / 上下限
  ThrustFilterMemory : UnitDelay  InitialCondition=single(0)  SampleTime=Official.Step
  UnusedStick{1..4,6} (5 alike) : Terminator
  UnusedStickMode : Terminator
  UnusedYaw : Terminator
  VerticalSpeedError : Sum  Inputs=+-
  VerticalSpeedPID : Subsystem  Description=速度誤差 → 推力補正
      mask Display: disp('鉛直速度 PID\n速度誤差 → 推力補正')
  YawRateError : Sum  Inputs=+-
  YawRatePID : Subsystem  Description=角速度誤差 → モーター差分
      mask Display: disp('Yaw 角速度 PID\n角速度誤差 → モーター差分')
  Zero : Constant  Value=single(0)
  Duty4 : Outport
  Counts4 : Outport  Port=2
  Diagnostics17 : Outport  Port=3
  AltFlag : Outport  Port=4
  FlipFlag : Outport  Port=5
  Reset : Outport  Port=6
  RateReference : Outport  Port=7
  FinalMode : Outport  Port=8
  wires:
  ControlDiagnosticPack/1(diag) -> [diag_S132P1]
  StickFields/5 -> [StickFields_S135P5]
  StickFields/6 -> [StickFields_S135P6]
  StickFields/4 -> [StickFields_S135P4]
  StickFields/3 -> [StickFields_S135P3]
  StickFields/2 -> [StickFields_S135P2]
  StickFields/1 -> [StickFields_S135P1]
  ResetAngles/1 -> [ResetAngles_S552P1]
  FlipAngleReset/1 -> [angleReset_S545P1]
  ControlEnableReset/8(flipFlag) -> [flipFlag_S127P8]
  LastRateReference/1 -> [LastRateReference_S551P1]
  ControlEnableReset/7(angleReset) -> [angleReset_S127P7]
  FinalizeFlightMode/1(mode) -> [mode_S553P1]
  ThrustFilterMemory/1 -> [ThrustFilterMemory_S133P1]
  HeldThrustMemory/1 -> [HeldThrustMemory_S134P1]
  ControlEnableReset/2(run) -> [run_S127P2]
  ControlEnableReset/3(reset) -> [reset_S127P3]
  ControlEnableReset/5(angleEnable) -> [angleEnable_S127P5]
  ControlEnableReset/4(altEnable) -> [altEnable_S127P4]
  ControlEnableReset/6(velEnable) -> [velEnable_S127P6]
  ResetPreviousAngles/1 -> [ResetPreviousAngles_S140P1]
  ResetPreviousAngles/2 -> [ResetPreviousAngles_S140P2]
  ControlEnableReset/1(command) -> [command_S127P1]
  [Stick6_S95P1] -> StickFields/1
  [height_S98P1] -> FinalizeFlightMode/3(height)
  [OverG_S102P1] -> FinalizeFlightMode/6(overG)
  [branch_S103P1] -> FinalizeFlightMode/1(branch)
  [branch_S103P1] -> ControlEnableReset/4(mode)
  [Dt_S104P1] -> ControlEnableReset/6(dt)
  [mode_S539P1] -> FinalizeFlightMode/2(preMode)
  [phase_S540P1] -> ControlEnableReset/9(phase)
  [thrust_S541P1] -> ControlEnableReset/10(flipThrust)
  [start_S543P1] -> FinalizeFlightMode/4(flipStart)
  [start_S543P1] -> ControlEnableReset/11(flipStart)
  [done_S544P1] -> FinalizeFlightMode/5(flipDone)
  [done_S544P1] -> ControlEnableReset/12(flipDone)
  [angleReset_S545P1] -> ResetAngles/3
  [Output_S149P1] -> ControlDiagnosticPack/4(zRef)
  [diag_S132P1] -> Diagnostics17/1
  [reset_S127P3] -> Reset/1
  [reset_S127P3] -> ResetAngles/1
  [angleReset_S127P7] -> ResetAngles/2
  [flipFlag_S127P8] -> FlipFlag/1
  [EstimatedAngles_S137P3] -> UnusedYaw/1
  [mode_S553P1] -> FinalMode/1
  [mode_S553P1] -> ControlEnableReset/13(finalMode)
  [HeldThrustMemory_S134P1] -> ControlEnableReset/8(lastThrust)
  [BeforeLimit4_S465P3] -> ControlDiagnosticPack/11(before)
  [Output_S374P1] -> ControlDiagnosticPack/9(pitchTorque)
  [Output_S329P1] -> ControlDiagnosticPack/8(rollTorque)
  [rate_S129P1] -> ControlDiagnosticPack/7(rate)
  [rate_S129P1] -> RateReference/1
  [rate_S129P1] -> LastRateReference/1
  [StickFields_S135P1] -> UnusedStick1/1
  [StickFields_S135P2] -> UnusedStick2/1
  [StickFields_S135P3] -> UnusedStick3/1
  [StickFields_S135P4] -> UnusedStick4/1
  [StickFields_S135P5] -> UnusedStickMode/1
  [StickFields_S135P6] -> UnusedStick6/1
  [angle_S128P1] -> ControlDiagnosticPack/6(angle)
  [resetError_S128P3] -> ResetPreviousAngles/1
  [alt_S126P1] -> ControlDiagnosticPack/1(alt)
  [base_S126P2] -> ControlDiagnosticPack/2(base)
  [counter_S126P3] -> ControlDiagnosticPack/3(counter)
  [raw_S126P4] -> ControlEnableReset/1(raw)
  [auto_S126P5] -> AltFlag/1
  [auto_S126P5] -> ControlEnableReset/3(auto)
  [manual_S126P6] -> ControlEnableReset/2(manual)
  [controlMode_S126P7] -> ControlEnableReset/5(controlMode)
  [thrust_S131P1] -> ControlDiagnosticPack/5(thrust)
  [filter_S131P2] -> ThrustFilterMemory/1
  [last_S131P3] -> HeldThrustMemory/1
  [ThrustFilterMemory_S133P1] -> ControlEnableReset/7(oldFilter)
  [Output_S419P1] -> ControlDiagnosticPack/10(yawTorque)
  [Zero_S141P1] -> AltitudePID/5(PreviousError)
  [Zero_S141P1] -> VerticalSpeedPID/5(PreviousError)
  [Zero_S141P1] -> RollRatePID/5(PreviousError)
  [Zero_S141P1] -> PitchRatePID/5(PreviousError)
  [Zero_S141P1] -> YawRatePID/5(PreviousError)
  [ThrustFilterMemory_S133P1] -> ThrustCorrectionLimits/9(oldFilter)
  [controlMode_S126P7] -> StickToAngleRate/10(controlMode)
  [manual_S126P6] -> ThrustCorrectionLimits/5(manual)
  [auto_S126P5] -> ThrustCorrectionLimits/4(auto)
  [auto_S126P5] -> SelectVerticalReference/3(auto)
  [base_S126P2] -> ThrustCorrectionLimits/3(base)
  [directRate_S128P2] -> SelectRateReference/1(direct)
  [ResetPreviousAngles_S140P2] -> PitchAnglePID/5(PreviousError)
  [ResetPreviousAngles_S140P1] -> RollAnglePID/5(PreviousError)
  [ResetAngles_S552P1] -> RollAnglePID/4(Reset)
  [ResetAngles_S552P1] -> PitchAnglePID/4(Reset)
  [LastRateReference_S551P1] -> StickToAngleRate/8(lastRate)
  [HeldThrustMemory_S134P1] -> ThrustCorrectionLimits/10(lastThrust)
  [mode_S553P1] -> SelectVerticalReference/2(mode)
  [flipFlag_S127P8] -> SelectVerticalReference/4(flipFlag)
  [flipFlag_S127P8] -> ThrustCorrectionLimits/11(flipFlag)
  [angleReset_S127P7] -> StickToAngleRate/7(angleReset)
  [velEnable_S127P6] -> VerticalSpeedPID/3(Enable)
  [velEnable_S127P6] -> ThrustCorrectionLimits/6(velEnable)
  [angleEnable_S127P5] -> RollAnglePID/3(Enable)
  [angleEnable_S127P5] -> SelectRateReference/4(angleEnable)
  [angleEnable_S127P5] -> PitchAnglePID/3(Enable)
  [altEnable_S127P4] -> AltitudePID/3(Enable)
  [reset_S127P3] -> RollRatePID/4(Reset)
  [reset_S127P3] -> StickToAngleRate/4(reset)
  [reset_S127P3] -> YawRatePID/4(Reset)
  [reset_S127P3] -> PitchRatePID/4(Reset)
  [reset_S127P3] -> MotorMixerFilter8bit/6(Reset)
  [reset_S127P3] -> AltitudePID/4(Reset)
  [reset_S127P3] -> VerticalSpeedPID/4(Reset)
  [run_S127P2] -> RollRatePID/3(Enable)
  [run_S127P2] -> StickToAngleRate/3(run)
  [run_S127P2] -> YawRatePID/3(Enable)
  [run_S127P2] -> MotorMixerFilter8bit/5(Run)
  [run_S127P2] -> PitchRatePID/3(Enable)
  [command_S127P1] -> ThrustCorrectionLimits/1(command)
  [done_S544P1] -> MotorMixerFilter8bit/10(HoldApplied)
  [done_S544P1] -> TakeoffLandingCommand/7(flipDone)
  [done_S544P1] -> StickToAngleRate/9(flipDone)
  [rollRate_S542P1] -> StickToAngleRate/6(flipRate)
  [phase_S540P1] -> StickToAngleRate/5(phase)
  [phase_S540P1] -> TakeoffLandingCommand/6(phase)
  [Dt_S104P1] -> PitchAnglePID/2(Dt)
  [Dt_S104P1] -> RollRatePID/2(Dt)
  [Dt_S104P1] -> AltitudePID/2(Dt)
  [Dt_S104P1] -> MotorMixerFilter8bit/9(Dt)
  [Dt_S104P1] -> ThrustCorrectionLimits/8(dt)
  [Dt_S104P1] -> VerticalSpeedPID/2(Dt)
  [Dt_S104P1] -> RollAnglePID/2(Dt)
  [Dt_S104P1] -> PitchRatePID/2(Dt)
  [Dt_S104P1] -> YawRatePID/2(Dt)
  [branch_S103P1] -> TakeoffLandingCommand/5(mode)
  [branch_S103P1] -> StickToAngleRate/2(mode)
  [branch_S103P1] -> MotorMixerFilter8bit/8(Mode)
  [branch_S103P1] -> ThrustCorrectionLimits/7(mode)
  [OverG_S102P1] -> MotorMixerFilter8bit/7(OverG)
  [RangeFlag_S101P1] -> TakeoffLandingCommand/4(rangeFlag)
  [Voltage_S100P1] -> TakeoffLandingCommand/3(voltage)
  [velocity_S99P1] -> VerticalSpeedError/2
  [height_S98P1] -> TakeoffLandingCommand/2(height)
  [height_S98P1] -> AltitudeError/2
  [gf_S97P1] -> EstimatedRates/1
  [a_S96P1] -> EstimatedAngles/1
  [Stick6_S95P1] -> TakeoffLandingCommand/1(stick)
  [Stick6_S95P1] -> StickToAngleRate/1(stick)
  FlipDone/1 -> [done_S544P1]
  OverG/1 -> [OverG_S102P1]
  TakeoffLandingCommand/3(counter) -> [counter_S126P3]
  RollRatePID/1(Output) -> MotorMixerFilter8bit/2(RollTorque), [Output_S329P1]
  ThrustCorrectionLimits/1(thrust) -> [thrust_S131P1], MotorMixerFilter8bit/1(Thrust)
  ThrustCorrectionLimits/3(last) -> [last_S131P3]
  ThrustCorrectionLimits/2(filter) -> [filter_S131P2]
  TakeoffLandingCommand/2(base) -> [base_S126P2]
  VerticalSpeedPID/1(Output) -> ThrustCorrectionLimits/2(correction)
  YawRateError/1 -> YawRatePID/1(Error)
  PitchRateError/1 -> PitchRatePID/1(Error)
  RollRateError/1 -> RollRatePID/1(Error)
  PitchAngleError/1 -> PitchAnglePID/1(Error)
  RollAngleError/1 -> RollAnglePID/1(Error)
  VerticalSpeedError/1 -> VerticalSpeedPID/1(Error)
  Zero/1 -> [Zero_S141P1]
  AltitudeError/1 -> AltitudePID/1(Error)
  EstimatedRates/3 -> YawRateError/2
  TargetRates/3 -> YawRateError/1
  EstimatedRates/2 -> PitchRateError/2
  TargetRates/2 -> PitchRateError/1
  EstimatedRates/1 -> RollRateError/2
  TargetRates/1 -> RollRateError/1
  Velocity/1 -> [velocity_S99P1]
  SelectVerticalReference/1(vRef) -> VerticalSpeedError/1
  TakeoffLandingCommand/1(alt) -> [alt_S126P1], AltitudeError/1
  AltitudePID/1(Output) -> [Output_S149P1], SelectVerticalReference/1(zRef)
  SelectRateReference/1(rate) -> TargetRates/1, [rate_S129P1]
  PitchAnglePID/1(Output) -> SelectRateReference/3(pitchPID)
  RollAnglePID/1(Output) -> SelectRateReference/2(rollPID)
  StickToAngleRate/2(directRate) -> [directRate_S128P2]
  Rates3/1 -> [gf_S97P1]
  Dt/1 -> [Dt_S104P1]
  TakeoffLandingCommand/5(auto) -> [auto_S126P5]
  TakeoffLandingCommand/6(manual) -> [manual_S126P6]
  TakeoffLandingCommand/4(raw) -> [raw_S126P4]
  Mode/1 -> [branch_S103P1]
  RangeFlag/1 -> [RangeFlag_S101P1]
  Voltage/1 -> [Voltage_S100P1]
  Height/1 -> [height_S98P1]
  Stick6/1 -> [Stick6_S95P1]
  FlipPhase/1 -> [phase_S540P1]
  FlipThrust/1 -> [thrust_S541P1]
  FlipStart/1 -> [start_S543P1]
  TakeoffLandingCommand/7(controlMode) -> [controlMode_S126P7]
  FlipRate/1 -> [rollRate_S542P1]
  PreMode/1 -> [mode_S539P1]
  EstimatedAngles/3 -> [EstimatedAngles_S137P3]
  StickToAngleRate/1(angle) -> [angle_S128P1], AngleTargets/1
  StickToAngleRate/3(resetError) -> [resetError_S128P3]
  Attitude3/1 -> [a_S96P1]
  AngleTargets/1 -> RollAngleError/1
  EstimatedAngles/1 -> RollAngleError/2
  AngleTargets/2 -> PitchAngleError/1
  EstimatedAngles/2 -> PitchAngleError/2
  PitchRatePID/1(Output) -> MotorMixerFilter8bit/3(PitchTorque), [Output_S374P1]
  YawRatePID/1(Output) -> [Output_S419P1], MotorMixerFilter8bit/4(YawTorque)
  MotorMixerFilter8bit/1(Duty4) -> Duty4/1
  MotorMixerFilter8bit/2(Counts4) -> Counts4/1
  MotorMixerFilter8bit/3(BeforeLimit4) -> [BeforeLimit4_S465P3]

== system StampFly_StudentBlocks/Controllers/VerticalSpeedPID ==
  Error : Inport
  Dt : Inport  Port=2
  Enable : Inport  Port=3
  Reset : Inport  Port=4
  PreviousError : Inport  Port=5
  ApplyKp : Product
  DMemory : UnitDelay  InitialCondition=single(0)  SampleTime=Official.Step
  DerivativeDenominator : Sum
  DerivativeErrorProduct : Product
  DerivativeErrorTerm : Product  Inputs=*/
  DerivativePreviousNumerator : Sum  Inputs=+-
  DerivativeUpdate : Sum
  DivideTi : Product  Inputs=*/
  EMemory : UnitDelay  InitialCondition=single(0)  SampleTime=Official.Step
  ErrorDifference : Sum  Inputs=+-
  ErrorPair : Sum
  ErrorPairDt : Product
  Eta : Constant  Value=single(0.125)
  EtaTd : Product
  HalfIntegral : Gain  Gain=single(.5)
  IMemory : UnitDelay  InitialCondition=single(0)  SampleTime=Official.Step
  IntegralLimit : Saturate  UpperLimit=single(30000)  LowerLimit=single(-30000)
  IntegralUpdate : Sum
  Kp : Constant  Value=single(0.0799999982)
  PIDTerms : Sum  Inputs=+++
  PreviousDerivativeProduct : Product
  PreviousDerivativeTerm : Product  Inputs=*/
  Select_dnext : Switch  Criteria=u2 ~= 0  SaturateOnIntegerOverflow=off  InputSameDT=off
  Select_dp : Switch  Criteria=u2 ~= 0  SaturateOnIntegerOverflow=off  InputSameDT=off
  Select_enext : Switch  Criteria=u2 ~= 0  SaturateOnIntegerOverflow=off  InputSameDT=off
  Select_ep : Switch  Criteria=u2 ~= 0  SaturateOnIntegerOverflow=off  InputSameDT=off
  Select_inext : Switch  Criteria=u2 ~= 0  SaturateOnIntegerOverflow=off  InputSameDT=off
  Select_ip : Switch  Criteria=u2 ~= 0  SaturateOnIntegerOverflow=off  InputSameDT=off
  Select_output : Switch  Criteria=u2 ~= 0  SaturateOnIntegerOverflow=off  InputSameDT=off
  Select_ynext : Switch  Criteria=u2 ~= 0  SaturateOnIntegerOverflow=off  InputSameDT=off
  Td : Constant  Value=single(0.0799999982)
  Ti : Constant  Value=single(0.949999988)
  TwiceEtaTd : Gain  Gain=single(2)
  TwiceTd : Gain  Gain=single(2)
  YMemory : UnitDelay  InitialCondition=single(0)  SampleTime=Official.Step
  Zero : Constant  Value=single(0)
  Output : Outport
  wires:
  Enable/1 -> Select_output/2, Select_inext/2, Select_dnext/2, Select_enext/2, Select_ynext/2
  ApplyKp/1 -> Select_ynext/1, Select_output/1
  YMemory/1 -> Select_ynext/3, Select_output/3
  Select_ynext/1 -> YMemory/1
  Select_output/1 -> Output/1
  Select_enext/1 -> EMemory/1
  Select_dnext/1 -> DMemory/1
  Select_inext/1 -> IMemory/1
  PIDTerms/1 -> ApplyKp/2
  Kp/1 -> ApplyKp/1
  DerivativeUpdate/1 -> PIDTerms/3, Select_dnext/1
  IntegralLimit/1 -> PIDTerms/2, Select_inext/1
  DerivativeErrorTerm/1 -> DerivativeUpdate/2
  PreviousDerivativeTerm/1 -> DerivativeUpdate/1
  DerivativeErrorProduct/1 -> DerivativeErrorTerm/1
  ErrorDifference/1 -> DerivativeErrorProduct/2
  TwiceTd/1 -> DerivativeErrorProduct/1
  DerivativeDenominator/1 -> PreviousDerivativeTerm/2, DerivativeErrorTerm/2
  PreviousDerivativeProduct/1 -> PreviousDerivativeTerm/1
  Select_dp/1 -> PreviousDerivativeProduct/2, Select_dnext/3
  DerivativePreviousNumerator/1 -> PreviousDerivativeProduct/1
  TwiceEtaTd/1 -> DerivativePreviousNumerator/1, DerivativeDenominator/1
  EtaTd/1 -> TwiceEtaTd/1
  Td/1 -> EtaTd/2, TwiceTd/1
  Eta/1 -> EtaTd/1
  IntegralUpdate/1 -> IntegralLimit/1
  DivideTi/1 -> IntegralUpdate/2
  Select_ip/1 -> Select_inext/3, IntegralUpdate/1
  Ti/1 -> DivideTi/2
  HalfIntegral/1 -> DivideTi/1
  ErrorPairDt/1 -> HalfIntegral/1
  ErrorPair/1 -> ErrorPairDt/2
  Dt/1 -> ErrorPairDt/1, DerivativeDenominator/2, DerivativePreviousNumerator/2
  Select_ep/1 -> Select_enext/3, ErrorPair/2, ErrorDifference/2
  Error/1 -> ErrorPair/1, ErrorDifference/1, PIDTerms/1, Select_enext/1
  EMemory/1 -> Select_ep/3
  PreviousError/1 -> Select_ep/1
  DMemory/1 -> Select_dp/3
  IMemory/1 -> Select_ip/3
  Reset/1 -> Select_ip/2, Select_dp/2, Select_ep/2
  Zero/1 -> Select_ip/1, Select_dp/1

== system StampFly_StudentBlocks/Controllers/YawRatePID ==
  Error : Inport
  Dt : Inport  Port=2
  Enable : Inport  Port=3
  Reset : Inport  Port=4
  PreviousError : Inport  Port=5
  ApplyKp : Product
  DMemory : UnitDelay  InitialCondition=single(0)  SampleTime=Official.Step
  DerivativeDenominator : Sum
  DerivativeErrorProduct : Product
  DerivativeErrorTerm : Product  Inputs=*/
  DerivativePreviousNumerator : Sum  Inputs=+-
  DerivativeUpdate : Sum
  DivideTi : Product  Inputs=*/
  EMemory : UnitDelay  InitialCondition=single(0)  SampleTime=Official.Step
  ErrorDifference : Sum  Inputs=+-
  ErrorPair : Sum
  ErrorPairDt : Product
  Eta : Constant  Value=single(0.125)
  EtaTd : Product
  HalfIntegral : Gain  Gain=single(.5)
  IMemory : UnitDelay  InitialCondition=single(0)  SampleTime=Official.Step
  IntegralLimit : Saturate  UpperLimit=single(30000)  LowerLimit=single(-30000)
  IntegralUpdate : Sum
  Kp : Constant  Value=single(3)
  PIDTerms : Sum  Inputs=+++
  PreviousDerivativeProduct : Product
  PreviousDerivativeTerm : Product  Inputs=*/
  Select_dnext : Switch  Criteria=u2 ~= 0  SaturateOnIntegerOverflow=off  InputSameDT=off
  Select_dp : Switch  Criteria=u2 ~= 0  SaturateOnIntegerOverflow=off  InputSameDT=off
  Select_enext : Switch  Criteria=u2 ~= 0  SaturateOnIntegerOverflow=off  InputSameDT=off
  Select_ep : Switch  Criteria=u2 ~= 0  SaturateOnIntegerOverflow=off  InputSameDT=off
  Select_inext : Switch  Criteria=u2 ~= 0  SaturateOnIntegerOverflow=off  InputSameDT=off
  Select_ip : Switch  Criteria=u2 ~= 0  SaturateOnIntegerOverflow=off  InputSameDT=off
  Select_output : Switch  Criteria=u2 ~= 0  SaturateOnIntegerOverflow=off  InputSameDT=off
  Select_ynext : Switch  Criteria=u2 ~= 0  SaturateOnIntegerOverflow=off  InputSameDT=off
  Td : Constant  Value=single(0.00999999978)
  Ti : Constant  Value=single(0.800000012)
  TwiceEtaTd : Gain  Gain=single(2)
  TwiceTd : Gain  Gain=single(2)
  YMemory : UnitDelay  InitialCondition=single(0)  SampleTime=Official.Step
  Zero : Constant  Value=single(0)
  Output : Outport
  wires:
  Enable/1 -> Select_output/2, Select_inext/2, Select_dnext/2, Select_enext/2, Select_ynext/2
  ApplyKp/1 -> Select_ynext/1, Select_output/1
  YMemory/1 -> Select_ynext/3, Select_output/3
  Select_ynext/1 -> YMemory/1
  Select_output/1 -> Output/1
  Select_enext/1 -> EMemory/1
  Select_dnext/1 -> DMemory/1
  Select_inext/1 -> IMemory/1
  PIDTerms/1 -> ApplyKp/2
  Kp/1 -> ApplyKp/1
  DerivativeUpdate/1 -> PIDTerms/3, Select_dnext/1
  IntegralLimit/1 -> PIDTerms/2, Select_inext/1
  DerivativeErrorTerm/1 -> DerivativeUpdate/2
  PreviousDerivativeTerm/1 -> DerivativeUpdate/1
  DerivativeErrorProduct/1 -> DerivativeErrorTerm/1
  ErrorDifference/1 -> DerivativeErrorProduct/2
  TwiceTd/1 -> DerivativeErrorProduct/1
  DerivativeDenominator/1 -> PreviousDerivativeTerm/2, DerivativeErrorTerm/2
  PreviousDerivativeProduct/1 -> PreviousDerivativeTerm/1
  Select_dp/1 -> PreviousDerivativeProduct/2, Select_dnext/3
  DerivativePreviousNumerator/1 -> PreviousDerivativeProduct/1
  TwiceEtaTd/1 -> DerivativePreviousNumerator/1, DerivativeDenominator/1
  EtaTd/1 -> TwiceEtaTd/1
  Td/1 -> EtaTd/2, TwiceTd/1
  Eta/1 -> EtaTd/1
  IntegralUpdate/1 -> IntegralLimit/1
  DivideTi/1 -> IntegralUpdate/2
  Select_ip/1 -> Select_inext/3, IntegralUpdate/1
  Ti/1 -> DivideTi/2
  HalfIntegral/1 -> DivideTi/1
  ErrorPairDt/1 -> HalfIntegral/1
  ErrorPair/1 -> ErrorPairDt/2
  Dt/1 -> ErrorPairDt/1, DerivativeDenominator/2, DerivativePreviousNumerator/2
  Select_ep/1 -> Select_enext/3, ErrorPair/2, ErrorDifference/2
  Error/1 -> ErrorPair/1, ErrorDifference/1, PIDTerms/1, Select_enext/1
  EMemory/1 -> Select_ep/3
  PreviousError/1 -> Select_ep/1
  DMemory/1 -> Select_dp/3
  IMemory/1 -> Select_ip/3
  Reset/1 -> Select_ip/2, Select_dp/2, Select_ep/2
  Zero/1 -> Select_ip/1, Select_dp/1
